simulink model "sanxiangnibiandianlu"  (R2025a)
settings: Solver=VariableStepAuto  StartTime=0.0  StopTime=0.1  RelTol=1e-3
libraries: spsThreePhaseSeriesRLCBranchLib x2, spsDCVoltageSourceLib x1, slpidlib x1, spsPLL3phLib x1, spsPWMGenerator2LevelLib x1, spsThreePhaseVIMeasurementLib x1, spsThreePhaseSourceLib x1, spsUniversalBridgeLib x1, sps_lib x1
settings Model: Creator=小鱼  LastModifiedBy=小鱼
settings SolverCC: ZeroCrossControl=DisableAll

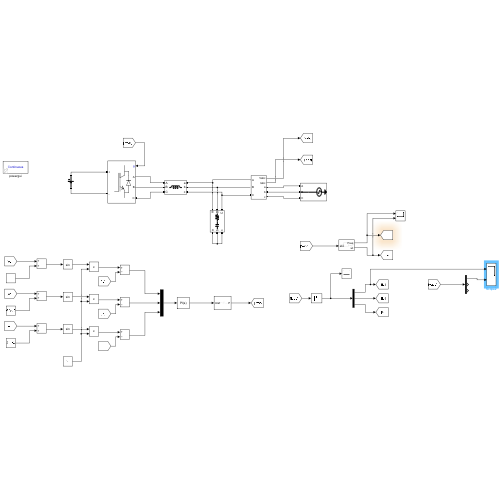
[thumbnail: Simulink's stored preview of the top-level diagram]
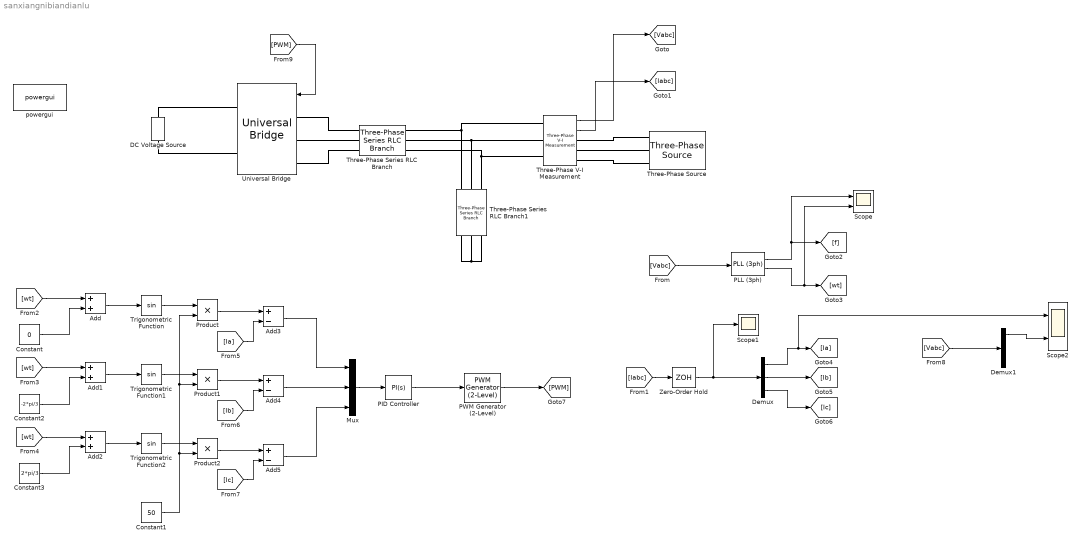
== system sanxiangnibiandianlu ==
  Add : Sum
  Add1 : Sum
  Add2 : Sum
  Add3 : Sum  Inputs=+-
  Add4 : Sum  Inputs=+-
  Add5 : Sum  Inputs=+-
  Constant : Constant  Value=0
  Constant1 : Constant  Value=50
  Constant2 : Constant  Value=-2*pi/3
  Constant3 : Constant  Value=2*pi/3
  DC Voltage Source : spsDCVoltageSourceLib/DC Voltage Source  Amplitude=600  Measurements=None
  Demux : Demux  Outputs=3
  Demux1 : Demux  Outputs=3
  Mux : Mux  Inputs=3
  PID Controller : slpidlib/PID Controller  Controller=PI  Form=Parallel  TimeDomain=Continuous-time  UseExternalTs=off  SampleTime=-1  IntegratorMethod=Forward Euler  FilterMethod=Forward Euler  ControllerParametersSource=internal  P=1  I=1  UseKiTs=off  D=0  UseExternalDerivativeSource=off  N=100  UseFilter=on  TunerSelectOption=Transfer Function Based (PID Tuner App)  InitialConditionSource=internal  InitialConditionForIntegrator=0  InitialConditionForFilter=0  DifferentiatorICPrevScaledInput=0  ExternalReset=none  TrackingMode=off  Kt=1  LimitOutput=off  SatLimitsSource=internal  UpperSaturationLimit=inf  LowerSaturationLimit=-inf  LinearizeAsGain=on  AntiWindupMode=none  Kb=1  LimitIntegrator=off  UpperIntegratorSaturationLimit=inf  LowerIntegratorSaturationLimit=-inf  POutMin=[]  POutMax=[]  IOutMin=[]  IOutMax=[]  DOutMin=[]  DOutMax=[]  NOutMin=[]  NOutMax=[]  SumOutMin=[]  SumOutMax=[]  SaturationOutMin=[]  SaturationOutMax=[]  PParamMin=[]  PParamMax=[]  IParamMin=[]  IParamMax=[]  DParamMin=[]  DParamMax=[]  NParamMin=[]  NParamMax=[]  KbParamMin=[]  KbParamMax=[]  KtParamMin=[]  KtParamMax=[]  KbOutMin=[]  KbOutMax=[]  KtOutMin=[]  KtOutMax=[]  IntegratorOutMin=[]  IntegratorOutMax=[]  FilterOutMin=[]  FilterOutMax=[]  SumI1OutMin=[]  SumI1OutMax=[]  SumI2OutMin=[]  SumI2OutMax=[]  SumI3OutMin=[]  SumI3OutMax=[]  SumI4OutMin=[]  SumI4OutMax=[]  SumDOutMin=[]  SumDOutMax=[]  DifferentiatorOutMin=[]  DifferentiatorOutMax=[]  FilterDiffOutCoefMin=[]  FilterDiffOutCoefMax=[]  ReciprocalOutMin=[]  ReciprocalOutMax=[]  SumDenOutMin=[]  SumDenOutMax=[]  SumNumOutMin=[]  SumNumOutMax=[]  DivideOutMin=[]  DivideOutMax=[]  UdiffTsProdOutMin=[]  UdiffTsProdOutMax=[]  NTsProdOutMin=[]  NTsProdOutMax=[]  UintegralTsProdOutMin=[]  UintegralTsProdOutMax=[]  UngainTsProdOutMin=[]  UngainTsProdOutMax=[]  ClampingZeroOutDataTypeStr=Inherit: Inherit via back propagation  ClampingZeroOutMin=[]  ClampingZeroOutMax=[]  FilterDenConstantOutDataTypeStr=Inherit: Inherit via back propagation  FilterDenConstantOutMin=[]  FilterDenConstantOutMax=[]  PCopyOutDataTypeStr=Inherit: Inherit via back propagation  PCopyOutMin=[]  PCopyOutMax=[]  NCopyOutDataTypeStr=Inherit: Inherit via back propagation  NCopyOutMin=[]  NCopyOutMax=[]  IntegratorContinuousStateAttributes=''  IntegratorStateMustResolveToSignalObject=off  IntegratorRTWStateStorageClass=Auto  FilterContinuousStateAttributes=''  FilterStateMustResolveToSignalObject=off  FilterRTWStateStorageClass=Auto  ParallelPVariant=InternalParameters  IdealPVariant=Disabled  IVariant=InternalParameters  DVariant=Disabled  IntegratorVariant=Continuous  SatVariant=Disabled  AWVariant=Passthrough  PCopyVariant=Disabled  TRVariant=Disabled  FdbkBlocksVariant=Forward  IdealPFdbkVariant=Disabled  SatFdbkVariant=Disabled  DerivativeFilterVariant=Disabled  NVariant=Disabled  NCopyVariant=Disabled_SignalSpec  FilterICVariant=Disabled  IntegratorICVariant=InternalICs  ExternalResetVariant=Disabled  TRSumVariant=Passthrough  SumFdbkVariant=Disabled  SumVariant=Sum_PI  TsampFilterVariant=InternalTs  TsampNgainVariant=Passthrough  TsampIntegralVariant=Disabled_SignalSpec  ExternalSaturationOutDataTypeStr=Inherit: Same as second input  DerivativeSourceVariant=Disabled  PreIntVariant=InternalPreInt
  PLL (3ph) : spsPLL3phLib/PLL (3ph)  Fmin=45  Par_Init=[0, 50]  ParK=[180, 3200, 1]  TcD=1e-4  MaxRateChangeFreq=12  FilterCutOffFreq=25  Ts=0  AGC=on
  PWM Generator (2-Level) : spsPWMGenerator2LevelLib/PWM Generator (2-Level)  ModulatorType=Three-phase bridge (6 pulses)  ModulatorMode=Unsynchronized  Fc=100*50  Pc=90  nF=27  MinMax="[ -1  1 ]"  SamplingTechnique=Natural  ModulatingSignals=off  m=0.8  Freq=60  Phase=0  Ts=0  ShowCarrierOutport=off
  Product : Product
  Product1 : Product
  Product2 : Product
  Scope : Scope  NumInputPorts=2
      settings: ActiveDisplayYMinimum=-31.511266125030225  ActiveDisplayYMaximum=81.952827213560383
  Scope1 : Scope
      settings: ActiveDisplayYMinimum=-10.212927788075859  ActiveDisplayYMaximum=12.531762150807253
  Scope2 : Scope  NumInputPorts=2
      settings: ActiveDisplayYMinimum=-453.80249057040686  ActiveDisplayYMaximum=436.64920251157855  DataLoggingVariableName=ScopeData2
  Three-Phase Series RLC Branch : spsThreePhaseSeriesRLCBranchLib/Three-Phase Series RLC Branch  LConnTagsString=A|B|C  RConnTagsString=A|B|C  BranchType=L  Resistance=1  Inductance=1e-3  Capacitance=1e-6  Measurements=None
  Three-Phase Series RLC Branch1 : spsThreePhaseSeriesRLCBranchLib/Three-Phase Series RLC Branch  LConnTagsString=A|B|C  RConnTagsString=A|B|C  BranchType=RC  Resistance=0.01  Inductance=1e-3  Capacitance=1e-4  Measurements=None
  Three-Phase V-I Measurement : spsThreePhaseVIMeasurementLib/Three-Phase V-I Measurement  VoltageMeasurement=phase-to-ground  SetLabelV=off  LabelV=Vabc  Vpu=off  VpuLL=off  CurrentMeasurement=yes  SetLabelI=off  LabelI=Iabc  Ipu=off  Pbase=100e6  Vbase=500e3  OutputType=Complex  PhasorSimulation=off  PSBequivalent=0
  Three-Phase Source : spsThreePhaseSourceLib/Three-Phase Source  InternalConnection=Yg  VoltagePhases=off  Voltage=380  PhaseAngle=0  Voltage_phases=[25e3 25e3 25e3]/sqrt(3)  PhaseAngles_phases=[0 -120 +120]  Frequency=50  NonIdealSource=on  SpecifyImpedance=off  Resistance=0  Inductance=0  ShortCircuitLevel=100e6  BaseVoltage=25e3  XRratio=7  BusType=swing  Pref=10e3  Qref=0  Prefabc=[10e3, 10e3, 10e3]  Qrefabc=[0, 0, 0]  Qmin=-inf  Qmax=inf
  Trigonometric Function : Trigonometry
  Trigonometric Function1 : Trigonometry
  Trigonometric Function2 : Trigonometry
  Universal Bridge : spsUniversalBridgeLib/Universal Bridge  Arms=3  SnubberResistance=1e5  SnubberCapacitance=inf  Device=IGBT / Diodes  Ron=1e-3  Lon=0  ForwardVoltages="[  0  0  ]"  ForwardVoltage=0  GTOparameters=[ 10e-6 , 20e-6 ]  IGBTparameters=[ 1e-6 , 2e-6 ]  Measurements=None  Measurements_2=None  converterType=Rectifier
  Zero-Order Hold : ZeroOrderHold  SampleTime=1e-5
  powergui : sps_lib/powergui  Priority=1  SimulationMode=Continuous  SampleTime=50e-6  frequency=60  Iterations=50  frequencyindice=50  Pbase=100e6  ErrMax=1e-4  UnitsV=kV  UnitsW=MW  buscounter=0  FunctionMessages=off  echomessages=off  EnableUseOfTLC=off  CurrentSourceSwitches=off  DisableSnubberDevices=off  DisableRonSwitches=off  DisableVfSwitches=off  DisplayEquations=off  AutomaticDiscreteSolvers=off  SolverType=Tustin/Backward Euler (TBE)  Interpol=off  ExternalGateDelay=off  methode=off  Ts=100  x0status=blocks  SPID=on  SwTol=0  HookPort=off  NonlinearTolerance=1e-4  nMaxIteration=100  ContinueOnMaxIteration=off  RestoreLinks=warning  ResistiveCurrentMeasurement=off  Frange=[0:2:500]  Ylog=off  Xlog=on  ShowGrid=off  save=off  variable=ZData  structure=0  ZoomFFT=off  StartTime=0.0  cycles=1  DisplayStyle=1  fundamental=60  FreqAxis=off  MaxFrequency=1000  frequencyindicesteady=1  RmsSteady=1  display=off
  wires:
  Three-Phase V-I Measurement/1 -> [Vabc]
  Three-Phase V-I Measurement/2 -> [Iabc]
  [Vabc] -> PLL (3ph)/1
  PLL (3ph)/1 -> Scope/1, [f]
  PLL (3ph)/2 -> Scope/2, [wt]
  [Iabc] -> Zero-Order Hold/1
  Demux/2 -> [Ib]
  Demux/3 -> [Ic]
  Demux/1 -> Scope2/1, [Ia]
  [wt] -> Add/1
  Constant/1 -> Add/2
  Add/1 -> Trigonometric Function/1
  Trigonometric Function/1 -> Product/1
  [wt] -> Add1/1
  Constant2/1 -> Add1/2
  Add1/1 -> Trigonometric Function1/1
  Trigonometric Function1/1 -> Product1/1
  Trigonometric Function2/1 -> Product2/1
  Add2/1 -> Trigonometric Function2/1
  [wt] -> Add2/1
  Constant3/1 -> Add2/2
  Constant1/1 -> Product2/2, Product1/2, Product/2
  Product/1 -> Add3/1
  Product1/1 -> Add4/1
  Product2/1 -> Add5/1
  [Ia] -> Add3/2
  [Ib] -> Add4/2
  [Ic] -> Add5/2
  Add4/1 -> Mux/2
  Add3/1 -> Mux/1
  Add5/1 -> Mux/3
  Mux/1 -> PID Controller/1
  PID Controller/1 -> PWM Generator (2-Level)/1
  PWM Generator (2-Level)/1 -> [PWM]
  Zero-Order Hold/1 -> Scope1/1, Demux/1
  [Vabc] -> Demux1/1
  Demux1/1 -> Scope2/2
  [PWM] -> Universal Bridge/1
  connections:
  DC Voltage Source/RConn1 -- Universal Bridge/RConn1
  DC Voltage Source/LConn1 -- Universal Bridge/RConn2
  Three-Phase Series RLC Branch/LConn2 -- Universal Bridge/LConn2
  Three-Phase Series RLC Branch/LConn1 -- Universal Bridge/LConn1
  Universal Bridge/LConn3 -- Three-Phase Series RLC Branch/LConn3
  Three-Phase Series RLC Branch1/LConn3 -- Three-Phase Series RLC Branch/RConn3 -- Three-Phase V-I Measurement/LConn3
  Three-Phase Series RLC Branch/RConn2 -- Three-Phase V-I Measurement/LConn2 -- Three-Phase Series RLC Branch1/LConn2
  Three-Phase Series RLC Branch1/LConn1 -- Three-Phase V-I Measurement/LConn1 -- Three-Phase Series RLC Branch/RConn1
  Three-Phase Source/RConn2 -- Three-Phase V-I Measurement/RConn2
  Three-Phase V-I Measurement/RConn1 -- Three-Phase Source/RConn1
  Three-Phase Source/RConn3 -- Three-Phase V-I Measurement/RConn3
  Three-Phase Series RLC Branch1/RConn1 -- Three-Phase Series RLC Branch1/RConn2 -- Three-Phase Series RLC Branch1/RConn3
